simulink model "BP_PID"  (R2024b)
settings: Solver=ode4  StartTime=0.0  StopTime=0.1  FixedStep=1e-7  RelTol=1e-3
libraries: spsSeriesRLCBranchLib x8, spsPWMGeneratorDCDCLib x4, spsVoltageMeasurementLib x3, spsControlledVoltageSourceLib x2, spsCurrentMeasurementLib x2, spsDiodeLib x2, spsGroundLib x2, spsIdealSwitchLib x2, spsMosfetLib x2, slpidlib x1, spspowerguiLib x1
settings Model: Creator=xjj  LastModifiedBy=xjj

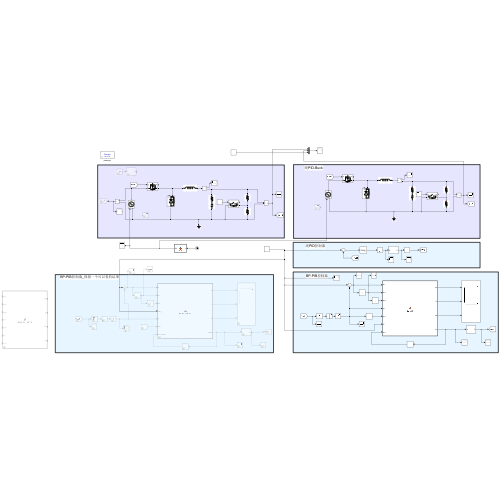
[thumbnail: Simulink's stored preview of the top-level diagram]
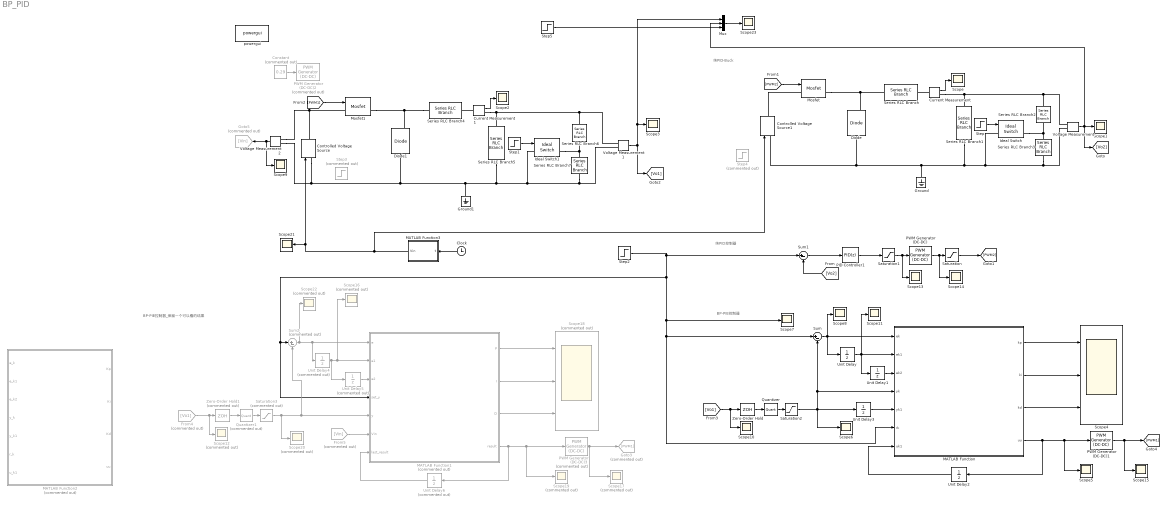
== system BP_PID ==
  note: BP-PIB控制器
  note: 纯PID-Buck
  note: 纯PID控制器
  note: BP-PIB控制器_保留一个可以看的结果
  Clock : Clock
  Constant : Constant  Commented=on  Value=0.29
  Controlled Voltage Source : spsControlledVoltageSourceLib/Controlled Voltage Source  Initialize=on  Source_Type=DC  Amplitude=42  Phase=0  Frequency=0  Measurements=None
  Controlled Voltage Source1 : spsControlledVoltageSourceLib/Controlled Voltage Source  Initialize=on  Source_Type=DC  Amplitude=42  Phase=0  Frequency=0  Measurements=None
  Current Measurement : spsCurrentMeasurementLib/Current Measurement  PhasorSimulation=off  OutputType=Complex  PSBequivalent=0
  Current Measurement1 : spsCurrentMeasurementLib/Current Measurement  PhasorSimulation=off  OutputType=Complex  PSBequivalent=0
  Diode : spsDiodeLib/Diode  Ron=0.001  Lon=0  Vf=0.8  IC=0  UseSnubber=0  Rs=500  Cs=250e-9  Measurements=on
  Diode1 : spsDiodeLib/Diode  Ron=0.001  Lon=0  Vf=0.8  IC=0  UseSnubber=0  Rs=500  Cs=250e-9  Measurements=on
  From4 : From  Commented=on  GotoTag=Vo1
  From5 : From  Commented=on  GotoTag=Vin
  Goto3 : Goto  Commented=on  GotoTag=PWM1
  Goto5 : Goto  Commented=on  GotoTag=Vin
  Ground : spsGroundLib/Ground  LConnTagsString=a
  Ground1 : spsGroundLib/Ground  LConnTagsString=a
  Ideal Switch : spsIdealSwitchLib/Ideal Switch  Ron=0.001  Lon=0  IC=1  Rs=1e5  Cs=inf  Measurements=on
  Ideal Switch1 : spsIdealSwitchLib/Ideal Switch  Ron=0.001  Lon=0  IC=1  Rs=1e5  Cs=inf  Measurements=on
  MATLAB Function : MATLAB Function  TreatAsAtomicUnit=on  SystemSampleTime=2e-5
  MATLAB Function1 : MATLAB Function  Commented=on  TreatAsAtomicUnit=on  SystemSampleTime=2e-5
  MATLAB Function2 : MATLAB Function  Commented=on  TreatAsAtomicUnit=on  SystemSampleTime=2e-5
  MATLAB Function3 : MATLAB Function  TreatAsAtomicUnit=on
  Mosfet : spsMosfetLib/Mosfet  Ron=0.1  Lon=0  Rd=0.01  Vfd=0  IC=0  Rs=1e5  Cs=inf  Measurements=on
  Mosfet1 : spsMosfetLib/Mosfet  Ron=0.1  Lon=0  Rd=0.01  Vfd=0  IC=0  Rs=1e5  Cs=inf  Measurements=on
  Mux : Mux  Inputs=3
  PID Controller1 : slpidlib/PID Controller  Controller=PID  Form=Parallel  TimeDomain=Discrete-time  UseExternalTs=off  SampleTime=-1  IntegratorMethod=Forward Euler  FilterMethod=Forward Euler  ControllerParametersSource=internal  P=0.02*8  I=50*2  UseKiTs=off  D=5e-5  UseExternalDerivativeSource=off  N=100  UseFilter=on  TunerSelectOption=Transfer Function Based (PID Tuner App)  InitialConditionSource=internal  InitialConditionForIntegrator=0  InitialConditionForFilter=0  DifferentiatorICPrevScaledInput=0  ExternalReset=none  TrackingMode=off  Kt=1  LimitOutput=off  SatLimitsSource=internal  UpperSaturationLimit=inf  LowerSaturationLimit=-inf  LinearizeAsGain=on  AntiWindupMode=none  Kb=1  LimitIntegrator=off  UpperIntegratorSaturationLimit=inf  LowerIntegratorSaturationLimit=-inf  POutMin=[]  POutMax=[]  IOutMin=[]  IOutMax=[]  DOutMin=[]  DOutMax=[]  NOutMin=[]  NOutMax=[]  SumOutMin=[]  SumOutMax=[]  SaturationOutMin=[]  SaturationOutMax=[]  PParamMin=[]  PParamMax=[]  IParamMin=[]  IParamMax=[]  DParamMin=[]  DParamMax=[]  NParamMin=[]  NParamMax=[]  KbParamMin=[]  KbParamMax=[]  KtParamMin=[]  KtParamMax=[]  KbOutMin=[]  KbOutMax=[]  KtOutMin=[]  KtOutMax=[]  IntegratorOutMin=[]  IntegratorOutMax=[]  FilterOutMin=[]  FilterOutMax=[]  SumI1OutMin=[]  SumI1OutMax=[]  SumI2OutMin=[]  SumI2OutMax=[]  SumI3OutMin=[]  SumI3OutMax=[]  SumI4OutMin=[]  SumI4OutMax=[]  SumDOutMin=[]  SumDOutMax=[]  DifferentiatorOutMin=[]  DifferentiatorOutMax=[]  FilterDiffOutCoefMin=[]  FilterDiffOutCoefMax=[]  ReciprocalOutMin=[]  ReciprocalOutMax=[]  SumDenOutMin=[]  SumDenOutMax=[]  SumNumOutMin=[]  SumNumOutMax=[]  DivideOutMin=[]  DivideOutMax=[]  UdiffTsProdOutMin=[]  UdiffTsProdOutMax=[]  NTsProdOutMin=[]  NTsProdOutMax=[]  UintegralTsProdOutMin=[]  UintegralTsProdOutMax=[]  UngainTsProdOutMin=[]  UngainTsProdOutMax=[]  ClampingZeroOutDataTypeStr=Inherit: Inherit via back propagation  ClampingZeroOutMin=[]  ClampingZeroOutMax=[]  FilterDenConstantOutDataTypeStr=Inherit: Inherit via back propagation  FilterDenConstantOutMin=[]  FilterDenConstantOutMax=[]  PCopyOutDataTypeStr=Inherit: Inherit via back propagation  PCopyOutMin=[]  PCopyOutMax=[]  NCopyOutDataTypeStr=Inherit: Inherit via back propagation  NCopyOutMin=[]  NCopyOutMax=[]  IntegratorContinuousStateAttributes=''  IntegratorStateMustResolveToSignalObject=off  IntegratorRTWStateStorageClass=Auto  FilterContinuousStateAttributes=''  FilterStateMustResolveToSignalObject=off  FilterRTWStateStorageClass=Auto  ParallelPVariant=InternalParameters  IdealPVariant=Disabled  IVariant=InternalParameters  DVariant=InternalParameters  IntegratorVariant=Discrete  SatVariant=Disabled  AWVariant=Passthrough  PCopyVariant=Disabled  TRVariant=Disabled  FdbkBlocksVariant=Forward  IdealPFdbkVariant=Disabled  SatFdbkVariant=Disabled  DerivativeFilterVariant=ForwardEulerFilter  NVariant=InternalParameters  NCopyVariant=Disabled  FilterICVariant=InternalICsFilter  IntegratorICVariant=InternalICs  ExternalResetVariant=Disabled  TRSumVariant=Passthrough  SumFdbkVariant=Disabled  SumVariant=Sum_PID  TsampFilterVariant=InternalTs  TsampNgainVariant=Passthrough  TsampIntegralVariant=Disabled_SignalSpec  ExternalSaturationOutDataTypeStr=Inherit: Same as second input  DerivativeSourceVariant=ErrorSignal  PreIntVariant=InternalPreInt
  PWM Generator (DC-DC) : spsPWMGeneratorDCDCLib/PWM Generator (DC-DC)  Fsw=50e3  Ts=0
  PWM Generator (DC-DC)1 : spsPWMGeneratorDCDCLib/PWM Generator (DC-DC)  Fsw=50e3  Ts=0
  PWM Generator (DC-DC)2 : spsPWMGeneratorDCDCLib/PWM Generator (DC-DC)  Commented=on  Fsw=50e3  Ts=0
  PWM Generator (DC-DC)3 : spsPWMGeneratorDCDCLib/PWM Generator (DC-DC)  Commented=on  Fsw=50e3  Ts=0
  Quantizer : Quantizer  QuantizationInterval=3.90625e-3
  Quantizer1 : Quantizer  Commented=on  QuantizationInterval=3.90625e-3
  Saturation : Saturate  UpperLimit=1  LowerLimit=0  ZeroCross=off
  Saturation1 : Saturate  UpperLimit=1  LowerLimit=0  ZeroCross=off
  Saturation2 : Saturate  UpperLimit=16  LowerLimit=0  ZeroCross=off
  Saturation3 : Saturate  Commented=on  UpperLimit=16  LowerLimit=0  ZeroCross=off
  Scope{,1..3,5..11,13..15,21,23} (16 alike) : Scope
  Scope{12,16..17,19..20,22} (6 alike) : Scope  Commented=on
  Scope18 : Scope  Commented=on  NumInputPorts=3
  Scope4 : Scope  NumInputPorts=3
  Series RLC Branch : spsSeriesRLCBranchLib/Series RLC Branch  LConnTagsString=__new0  RConnTagsString=__new0  BranchType=L  Resistance=0  Inductance=470e-6  SetiL0=off  InitialCurrent=0  Capacitance=inf  Setx0=off  InitialVoltage=0  Measurements=None
  Series RLC Branch1 : spsSeriesRLCBranchLib/Series RLC Branch  LConnTagsString=__new0  RConnTagsString=__new0  BranchType=RC  Resistance=0.1  Inductance=1e-3  SetiL0=off  InitialCurrent=0  Capacitance=220e-6  Setx0=off  InitialVoltage=0  Measurements=None
  Series RLC Branch2 : spsSeriesRLCBranchLib/Series RLC Branch  LConnTagsString=__new0  RConnTagsString=__new0  BranchType=R  Resistance=6  Inductance=1e-3  SetiL0=off  InitialCurrent=0  Capacitance=1e-6  Setx0=off  InitialVoltage=0  Measurements=None
  Series RLC Branch3 : spsSeriesRLCBranchLib/Series RLC Branch  LConnTagsString=__new0  RConnTagsString=__new0  BranchType=R  Resistance=54  Inductance=1e-3  SetiL0=off  InitialCurrent=0  Capacitance=1e-6  Setx0=off  InitialVoltage=0  Measurements=None
  Series RLC Branch4 : spsSeriesRLCBranchLib/Series RLC Branch  LConnTagsString=__new0  RConnTagsString=__new0  BranchType=L  Resistance=0  Inductance=470e-6  SetiL0=off  InitialCurrent=0  Capacitance=inf  Setx0=off  InitialVoltage=0  Measurements=None
  Series RLC Branch5 : spsSeriesRLCBranchLib/Series RLC Branch  LConnTagsString=__new0  RConnTagsString=__new0  BranchType=RC  Resistance=0.005*2*2*2  Inductance=1e-3  SetiL0=off  InitialCurrent=0  Capacitance=220e-6  Setx0=off  InitialVoltage=0  Measurements=None
  Series RLC Branch6 : spsSeriesRLCBranchLib/Series RLC Branch  LConnTagsString=__new0  RConnTagsString=__new0  BranchType=R  Resistance=6  Inductance=1e-3  SetiL0=off  InitialCurrent=0  Capacitance=1e-6  Setx0=off  InitialVoltage=0  Measurements=None
  Series RLC Branch7 : spsSeriesRLCBranchLib/Series RLC Branch  LConnTagsString=__new0  RConnTagsString=__new0  BranchType=R  Resistance=54  Inductance=1e-3  SetiL0=off  InitialCurrent=0  Capacitance=1e-6  Setx0=off  InitialVoltage=0  Measurements=None
  Step : Step  Time=0.08  Before=1  After=0  SampleTime=0  ZeroCross=off
  Step1 : Step  Time=0.08  Before=1  After=0  SampleTime=0  ZeroCross=off
  Step2 : Step  Time=0.001  After=12  SampleTime=2e-5  ZeroCross=off
  Step3 : Step  Commented=on  Time=0.03  Before=42  After=52  SampleTime=0
  Step4 : Step  Commented=on  Time=0.03  Before=42  After=52  SampleTime=0
  Step5 : Step  Time=0.001  After=12  SampleTime=2e-5  ZeroCross=off
  Sum : Sum  Inputs=|+-
  Sum1 : Sum  Inputs=|+-
  Sum2 : Sum  Commented=on  Inputs=|+-
  Unit Delay{,1..3} (4 alike) : UnitDelay  SampleTime=2e-5  HasFrameUpgradeWarning=on
  Unit Delay4 : UnitDelay  Commented=on  SampleTime=2e-5  HasFrameUpgradeWarning=on
  Unit Delay5 : UnitDelay  Commented=on  SampleTime=2e-5  HasFrameUpgradeWarning=on
  Unit Delay6 : UnitDelay  Commented=on  SampleTime=2e-5  HasFrameUpgradeWarning=on
  Voltage Measurement : spsVoltageMeasurementLib/Voltage Measurement  PhasorSimulation=off  OutputType=Complex  PSBequivalent=0
  Voltage Measurement1 : spsVoltageMeasurementLib/Voltage Measurement  PhasorSimulation=off  OutputType=Complex  PSBequivalent=0
  Voltage Measurement2 : spsVoltageMeasurementLib/Voltage Measurement  PhasorSimulation=off  OutputType=Complex  PSBequivalent=0
  Zero-Order Hold : ZeroOrderHold  SampleTime=2e-5
  Zero-Order Hold1 : ZeroOrderHold  Commented=on  SampleTime=2e-5
  powergui : spspowerguiLib/powergui  Priority=1  SimulationMode=Discrete  SampleTime=1e-7  frequency=60  Iterations=50  frequencyindice=0  Pbase=100e6  ErrMax=1e-4  UnitsV=kV  UnitsW=MW  buscounter=0  FunctionMessages=off  echomessages=off  EnableUseOfTLC=off  CurrentSourceSwitches=off  DisableSnubberDevices=off  DisableRonSwitches=off  DisableVfSwitches=off  DisplayEquations=off  AutomaticDiscreteSolvers=off  SolverType=Tustin/Backward Euler (TBE)  Interpol=off  ExternalGateDelay=off  methode=off  Ts=100  x0status=blocks  SPID=on  SwTol=0  HookPort=off  NonlinearTolerance=1e-4  nMaxIteration=100  ContinueOnMaxIteration=off  RestoreLinks=warning  ResistiveCurrentMeasurement=off  Frange=[0:2:500]  Ylog=off  Xlog=on  ShowGrid=off  save=off  variable=ZData  structure=0  ZoomFFT=off  StartTime=0.0  cycles=1  DisplayStyle=1  fundamental=60  FreqAxis=off  MaxFrequency=1000  frequencyindicesteady=1  RmsSteady=1  display=off
  wires:
  Current Measurement/1 -> Scope/1
  Voltage Measurement/1 -> Mux/2, [Vo2], Scope1/1
  Step/1 -> Ideal Switch/1
  Step2/1 -> MATLAB Function/6(rk), Sum/1, Scope7/1, MATLAB Function1/4(set_y), Sum2/1, Sum1/1
  [Vo2] -> Sum1/2
  Sum1/1 -> PID Controller1/1
  PID Controller1/1 -> Saturation1/1
  Saturation1/1 -> Scope13/1, PWM Generator (DC-DC)/1
  PWM Generator (DC-DC)/1 -> Scope14/1, Saturation/1
  Saturation/1 -> [PWM2]
  [PWM2] -> Mosfet/1
  Voltage Measurement1/1 -> [Vo1], Mux/1, Scope3/1
  Current Measurement1/1 -> Scope2/1
  [Vo1] -> Scope10/1, Zero-Order Hold/1
  Zero-Order Hold/1 -> Quantizer/1
  Quantizer/1 -> Saturation2/1
  Saturation2/1 -> Unit Delay3/1, MATLAB Function/4(yk), Sum/2, Scope6/1
  Sum/1 -> MATLAB Function/1(ek), Unit Delay/1, Scope8/1
  Unit Delay/1 -> MATLAB Function/2(ek1), Scope11/1, Unit Delay1/1
  Voltage Measurement2/1 -> Goto5/1, Scope9/1
  MATLAB Function/1(kp) -> Scope4/1
  MATLAB Function/2(ki) -> Scope4/2
  MATLAB Function/3(kd) -> Scope4/3
  MATLAB Function/4(uu) -> PWM Generator (DC-DC)1/1, Scope5/1, Unit Delay2/1
  PWM Generator (DC-DC)1/1 -> [PWM1], Scope15/1
  Unit Delay1/1 -> MATLAB Function/3(ek2)
  Unit Delay2/1 -> MATLAB Function/7(uk1)
  Constant/1 -> PWM Generator (DC-DC)2/1
  [PWM1] -> Mosfet1/1
  PWM Generator (DC-DC)3/1 -> Goto3/1, Scope17/1
  Sum2/1 -> Unit Delay4/1, MATLAB Function1/1(e), Scope22/1
  Unit Delay5/1 -> MATLAB Function1/3(e2)
  Unit Delay6/1 -> MATLAB Function1/7(last_result)
  From4/1 -> Scope12/1, Zero-Order Hold1/1
  Quantizer1/1 -> Saturation3/1
  Zero-Order Hold1/1 -> Quantizer1/1
  MATLAB Function1/3(D) -> Scope18/3
  Saturation3/1 -> MATLAB Function1/5(y), Sum2/2, Scope20/1
  MATLAB Function1/2(I) -> Scope18/2
  MATLAB Function1/1(P) -> Scope18/1
  MATLAB Function1/4(result) -> Scope19/1, PWM Generator (DC-DC)3/1, Unit Delay6/1
  Unit Delay4/1 -> MATLAB Function1/2(e1), Scope16/1, Unit Delay5/1
  From5/1 -> MATLAB Function1/6(Vin)
  Unit Delay3/1 -> MATLAB Function/5(yk1)
  Clock/1 -> MATLAB Function3/1(t)
  MATLAB Function3/1(Vin) -> Controlled Voltage Source1/1, Controlled Voltage Source/1, Scope21/1
  Step1/1 -> Ideal Switch1/1
  Mux/1 -> Scope23/1
  Step5/1 -> Mux/3
  connections:
  Controlled Voltage Source1/RConn1 -- Mosfet/LConn1
  Mosfet/RConn1 -- Diode/RConn1 -- Series RLC Branch/LConn1
  Ideal Switch/LConn1 -- Voltage Measurement/LConn2 -- Series RLC Branch3/RConn1 -- Series RLC Branch1/RConn1 -- Ground/LConn1 -- Controlled Voltage Source1/LConn1 -- Diode/LConn1
  Series RLC Branch2/LConn1 -- Voltage Measurement/LConn1 -- Current Measurement/RConn1 -- Series RLC Branch1/LConn1
  Current Measurement/LConn1 -- Series RLC Branch/RConn1
  Series RLC Branch3/LConn1 -- Ideal Switch/RConn1 -- Series RLC Branch2/RConn1
  Series RLC Branch4/LConn1 -- Mosfet1/RConn1 -- Diode1/RConn1
  Series RLC Branch5/LConn1 -- Voltage Measurement1/LConn1 -- Series RLC Branch6/LConn1 -- Current Measurement1/RConn1
  Series RLC Branch6/RConn1 -- Series RLC Branch7/LConn1 -- Ideal Switch1/RConn1
  Mosfet1/LConn1 -- Voltage Measurement2/LConn1 -- Controlled Voltage Source/RConn1
  Current Measurement1/LConn1 -- Series RLC Branch4/RConn1
  Diode1/LConn1 -- Controlled Voltage Source/LConn1 -- Voltage Measurement2/LConn2 -- Voltage Measurement1/LConn2 -- Series RLC Branch7/RConn1 -- Ideal Switch1/LConn1 -- Series RLC Branch5/RConn1 -- Ground1/LConn1

== matlab function BP_PID/MATLAB Function1 ==
  data: e input; P output; e1 input; e2 input; set_y input; y input; Vin input; last_result input; I output; D output; result output
function [P,I,D,result] = my_bp_pid_fcn(e, e1, e2, set_y, y, Vin, last_result)
% BP‑PID自适应控制器
% 网络：输入层[set_y,e,y] 3神经元；隐含层5神经元Tanh；输出层[P,I,D] 3神经元Sigmoid
% 输出：P,I,D（PID参数），result（限幅后的占空比）

if any(isnan([e, e1, e2, set_y, y, Vin, last_result]))
    warning('Input contains NaN!');
end

persistent w1 w2 
persistent dw2 dw1

%% =========权重初始化，仅首次运行执行=========
if isempty(w1)
    w1 = 0.1 * randn(5,3); % 输入层(3) → 隐含层(5)
    w2 = 0.1 * randn(3,5); % 隐含层(5) → 输出层(3)
    
    dw1 = zeros(size(w1));
    dw2 = zeros(size(w2));
end

%% =========【BP正向传播】=========
x = [set_y/12; e/12; y/12];
% 倘若输入归一化
%x = [set_y / Vin; e / Vin; y / Vin];

% 输入层→隐含层
h_in = w1 * x;
h_out = (exp(h_in) - exp(-h_in)) ./ (exp(h_in) + exp(-h_in)); % Tanh激活

% 隐含层→输出层
o_in = w2 * h_out;
o_out = exp(o_in) ./ (exp(o_in) + exp(-o_in)); % Sigmoid激活（保证PID参数>0）

kp = 10;
ki = 5;
kd = 1;

P = kp * o_out(1);
I = ki * o_out(2);
D = kd * o_out(3);

% 尝试看看PID
% disp()

%% =========增量式PID计算占空比=========
delta_e1 = e - e1;
delta_e2 = e - 2*e1 + e2;
delta_u  = P * delta_e1 + I * e + D * delta_e2;
%delta_u  = 10 *P * delta_e1 + 5 * I * e + D * delta_e2;

u_k = last_result + delta_u;

result = sat_limit(u_k, 0, 1); 
%result = u_k;

%% =========【反向传播，严格按PPT（无偏置，带Momentum）】=========
eta   = 0.15;    % 学习速率
alpha = 0.3;   % 动量因子

%  损失函数求导 
% E = 0.5 * (set_y - y)^2

dE_dy = -e;

%  系统模型导数 dy/du 
% 占空比到实际输出电压的导数。如果无法建模，可设为常数1，或近似为 (y_k - y_prev)/(u_k - u_prev)
dy_du = 1; 
% dy_du = Vin; 

%  输出层梯度计算（链式求导）
% 增量式PID：u = P*Δe1 + I*e + D*Δe2
% 所以 ∂u/∂P = Δe1,  ∂u/∂I = e,  ∂u/∂D = Δe2
dU_dPID = [kp * delta_e1; ki * e; kd * delta_e2];

% 平移tanh导数：O' = 2 * O .* (1 - O)
dO_dw2H = 2* o_out .* (1 - o_out);

% 先对w2求偏导 优先更新w2权重网络
dw2H_dw2 = h_out;

% 先更新w2权重
% 保存一下旧的w2 用旧的w2更新w1
w2_last = w2;
% 得出损失函数对w2的偏导
dE_dw2 = ((dE_dy * dy_du) * dU_dPID .* dO_dw2H) * dw2H_dw2';
dw2_last = dw2;
dw2 = -eta * dE_dw2 + alpha * dw2_last;
w2 = w2 + dw2;

% 继续反向传播
%dw2H_dH = w2;
dw2H_dH = w2_last;

% 对隐藏层的激活函数tanh求偏导
dH_w1x = 1 - h_out.^2;

dw1x_dw1 = x;

% 更新w1权重
%得出损失函数对w1的梯度
dE_dw1 = ((dw2H_dH' * ((dE_dy * dy_du) * dU_dPID .* dO_dw2H)) .* dH_w1x) * dw1x_dw1';
dw1_last = dw1;
dw1 = -eta * dE_dw1 + alpha * dw1_last;
w1 = w1 + dw1;

%disp([P, I, D, result])

end

%% 子函数：饱和限幅
function y = sat_limit(x, low, high)
y = x;
y(x < low)  = low;
y(x > high) = high;
end

== matlab function BP_PID/MATLAB Function ==
  data: ek input; kp output; ek1 input; ek2 input; yk input; yk1 input; rk input; uk1 input; ki output; kd output; uu output
function [kp, ki, kd, uu] = bp_pid(ek, ek1, ek2, yk, yk1, rk, uk1)
% BP 神经网络自整定增量式 PID (3-5-3)，已做电压归一化 + 增益缩放
%
%   接口:
%     输入 [ek ek1 ek2 yk yk1 rk uk1]  (原始物理量: 电压V、占空比)
%     输出 [kp ki kd uu]
%
%   NN 结构: 输入层3(rk,yk,ek) -> 隐含层5 -> 输出层3(Kp,Ki,Kd)
%   增量式PID: uu = uk1 + kp*(en-en1) + ki*en + kd*(en-2en1+en2)
%   反向传播: 梯度下降 + 动量，在线调整权值 wi/wo

persistent wi wo d_wi d_wo inited

% coder.extrinsic('assignin');

% ================= 可调参数 =================
xite = 0.002;   % 学习因子 (调小: 让NN增益变化更平滑，减少占空比抖动)
alfa = 0.05;    % 动量因子 (调大: 平滑权值更新，进一步减少抖动)
Vn   = 12.0;    % 电压归一化基准 (= 期望输出电压 rk)
Kps  = 0.015*2*2*2*2*2*2*2*2*2*2*2*2*2*2;   % Kp 增益缩放系数 (增量式PID中=阻尼项，抑制超调)
Kis  = 0.003*2*2*2*2*2*2*2*2*2*2*2*2;   % Ki 增益缩放系数 (增量式PID中=比例/提速项，兼顾速度与纹波)
Kds  = 0.0001*2*2*2*2*2*2*2*2;     % Kd 增益缩放系数 (二阶差分项在轻载时反阻尼，建议=0)
% ===========================================

use_pretrain = false;
if isempty(inited)
    if use_pretrain
        wi = [  -0.0414847786512617	-0.203834046977469	-0.0403951794390325
                0.110117471291384	-0.156886450982033	0.0925815314395502
                -0.249930909715862	-0.0772266509362417	-0.147754957801011
                -0.0987801729433129	-0.0515949747720053	0.189090970823578
                -0.176670516162666	0.0193911481119876	-0.236337446082566];
        wo = [  0.0852224277454449	-0.179783682089841	0.234084743010971	0.188203824564264	-0.230519193209343
                -0.0413765886581459	-0.150943181062454	-0.0933404046486878	0.197292910729872	-0.165122030484067
                0.0293449142228758	0.150372284337768	0.0961613078346570	-0.207477894315111	0.189071251714707];
    else
        rng(1);                       % 固定随机种子，保证每次初始化一致
        wi   = 0.5*rand(5,3) - 0.25;  % 输入层->隐含层 权值 (5x3)
        wo   = 0.5*rand(3,5) - 0.25;  % 隐含层->输出层 权值 (3x5)
    end
    d_wi = zeros(5,3);
    d_wo = zeros(3,5);
    inited = 1;
end

% ---------- 归一化 (原始量 -> ~[0,1]) ----------
rn  = rk / Vn;    % 期望输出归一化
yn  = yk / Vn;    % 实际输出归一化
en  = ek / Vn;    % 当前误差归一化  (en = rn - yn)
en1 = ek1 / Vn;   % e(k-1) 归一化
en2 = ek2 / Vn;   % e(k-2) 归一化

% ---------- 正向传播 ----------
x  = [rn; yn; en];                  % 输入层 (3x1)
Oh = tanh(wi * x);                  % 隐含层输出 (5x1)
K  = 1 ./ (1 + exp(-2*(wo * Oh)));  % 输出层 (3x1)，Kp/Ki/Kd 落在 (0,1)
kp = Kps * K(1);  ki = Kis * K(2);  kd = Kds * K(3);

% ---------- 增量式 PID (在归一化误差上进行) ----------
du = kp*(en - en1) + ki*en + kd*(en - 2*en1 + en2);
uu = uk1 + du;
if uu < 0.05, uu = 0.05; end   % 占空比下限
if uu > 0.90, uu = 0.90; end   % 占空比上限

% ---------- 反向传播 (在线调整权值) ----------
dyu = 1;   % Buck: 占空比增大 -> 输出电压增大，dy/du 恒为正，取雅可比符号=+1

ddu = [Kps*(en - en1); Kis*en; Kds*(en - 2*en1 + en2)];  % du/d[K1,K2,K3] (3x1)
delta3 = en * dyu * ddu .* (2*K.*(1-K));                 % 输出层误差 (3x1)

d_wo = xite * (delta3 * Oh') + alfa * d_wo;              % 输出层权值修正 (3x5)
wo   = wo + d_wo;

delta2 = (1 - Oh.^2) .* (wo' * delta3);                  % 隐含层误差 (5x1)
d_wi   = xite * (delta2 * x') + alfa * d_wi;             % 隐含层权值修正 (5x3)
wi     = wi + d_wi;

% assignin('base', 'wi_final', wi);
% assignin('base', 'wo_final', wo);

end

== matlab function BP_PID/MATLAB Function2 ==
  data: e_k input; Kp output; e_k1 input; e_k2 input; y_k input; y_k1 input; r_k input; u_k1 input; Ki output; Kd output; uu output
function [Kp, Ki, Kd, uu] = github_bp_pid_fcn(e_k, e_k1, e_k2, y_k, y_k1, r_k, u_k1)
% BP-PID 控制器 (3-5-3)
% 输入: e_k, e_k1, e_k2, y_k, y_k1, r_k, u_k1  (均为标量)
% 输出: Kp, Ki, Kd, uu

% ================= 可调参数 =================
nh    = 5;        % 隐含层节点数
xite  = 0.02;     % 学习率
alfa  = 0.05;     % 动量因子

% PID 参数范围（保证非零）
Kp_min = 0.5;  Kp_max = 12;
Ki_min = 0.05; Ki_max = 1.2;
Kd_min = 0.05; Kd_max = 0.5;

% 误差限幅
E_MAX = 5;

% 控制量（占空比/电压）输出范围
%   PWM 占空比 → [0, 1]
%   电压输出  → [0, 12]（你的系统）
UU_MIN = 0;
UU_MAX = 12;

% ================= persistent 权值 =================
persistent wi_1 wo_1 wi_2 wo_2
if isempty(wi_1)
    rng(0);   % 固定种子，便于复现
    wi_1 = (rand(nh,3)-0.5)*0.5;   % 5×3
    wo_1 = (rand(3,nh)-0.5)*0.5;   % 3×5
    wi_2 = wi_1;  wo_2 = wo_1;
end

% ================= 1. 输入限幅 =================
e_k  = max(min(e_k,  E_MAX), -E_MAX);
e_k1 = max(min(e_k1, E_MAX), -E_MAX);
e_k2 = max(min(e_k2, E_MAX), -E_MAX);

% ================= 2. 网络输入 =================
xi = [r_k, y_k, e_k];
xx = [e_k-e_k1; e_k; e_k+e_k2-2*e_k1];
xx = max(min(xx, E_MAX), -E_MAX);

% ================= 3. 前向传播 =================
I  = xi * wi_1';                    % 1×5
Oh = 1 ./ (1 + exp(-2*I));          % 1×5 (Sigmoid)

O  = wo_1 * Oh';                    % 3×1
s  = 1 ./ (1 + exp(-O));            % Sigmoid，值域 (0,1)

% 关键：用 sigmoid 映射到 [Kmin, Kmax]，K 永远不会是 0
Kmin = [Kp_min; Ki_min; Kd_min];
Kmax = [Kp_max; Ki_max; Kd_max];
K    = Kmin + (Kmax - Kmin) .* s;   % 3×1，Kp/Ki/Kd 恒为正

% ================= 4. 增量式 PID =================
uu_raw = u_k1 + K' * xx;
uu     = max(min(uu_raw, UU_MAX), UU_MIN);

% % ================= 5. 反向传播 =================
dyu = sign((y_k - y_k1) / (uu - u_k1 + 1e-6));
if dyu == 0
    dyu = 1;    % 启动时 y 未变化，兜底为 +1 让权值能更新
end

dK_dO  = (Kmax - Kmin) .* s .* (1 - s);        % 3×1
delta3 = e_k * dyu * xx .* dK_dO;              % 3×1
delta3 = max(min(delta3, 0.5), -0.5);          % 梯度裁剪

wo = wo_1 + xite*delta3*Oh + alfa*(wo_1-wo_2);
wo = max(min(wo, 2), -2);                      % 权值限幅

dOh = 2 * Oh .* (1 - Oh);                      % 1×5
wi  = wi_1 + xite*(dOh .* (delta3'*wo))' * xi + alfa*(wi_1-wi_2);
wi  = max(min(wi, 2), -2);

% ================= 6. 保存权值 =================
wi_2 = wi_1;  wo_2 = wo_1;
wi_1 = wi;    wo_1 = wo;

% ================= 7. 输出 =================
Kp = K(1);
Ki = K(2);
Kd = K(3);
end

== matlab function BP_PID/MATLAB Function3 ==
  data: t input; Vin output
function Vin = clock(t)

if t<0.03
    Vin = 32;
elseif t>=0.03 && t<0.06
    Vin = 52;
else
    Vin = 42;
end
